simulink model "FinalSolution"  (R2025b)
settings: Solver=VariableStepAuto  StartTime=0.0  StopTime=0.8  FixedStep=SPWM_Ts  RelTol=1e-3
model workspace (MAT data in the model file):
  AC_LoadResistance = 9.23760430703
  AD_TimeConstant = 0.00025
  AD_a = [1 -0.881765205117]
  AD_b = [2.95586987209 -2.95586987209]
  CL_AAComp = 1.00249999972
  CL_Kaw = 20
  CL_Ki = 1.6
  CL_Kp = 0.005
  CL_N = 200
  CL_Ts = 0.0001
  CL_Vref = 32
  CL_faa = 1000
  CL_fp = 50
  CL_mff = 0.94
  CL_mmax = 1
  CommonModeBias = 0.15
  CommonModeKp = 0.02
  CommonModeShift = 1
  ControlStartTime = 0.06
  DampingCapuF = 4.7
  DampingResistance = 30
  DeadtimeComp = 0.08
  DeadtimeCurrentBand = 0.2
  DutyFeedforward = 0
  DutyMax = 0.75
  FilterDCR = 0.3
  KiCurrentLoop = 5
  KiVoltageLoop = 5
  KpCurrentLoop = 0.08
  KpVoltageLoop = 0.2
  LoadConnectTime = 0.18
  MainFilterCapuF = 4.7
  PR_Gain = 1.25
  PR_a10 = [1 -1.99838562653 0.999372033695]
  PR_a11 = [1 -1.99817857535 0.999372066214]
  PR_a13 = [1 -1.99770539603 0.999372140529]
  PR_a16 = [1 -1.99684804391 0.99937227518]
  PR_a17 = [1 -1.99652293757 0.99937232624]
  PR_a19 = [1 -1.9958137982 0.999372437614]
  PR_a2 = [1 -1.99933241937 0.999371884997]
  PR_a4 = [1 -1.99921404574 0.999371903588]
  PR_a5 = [1 -1.99912527012 0.99937191753]
  PR_a7 = [1 -1.9988885544 0.999371954708]
  PR_a8 = [1 -1.99874062131 0.999371977941]
  PR_b10 = [0.236875635534 -0.472442728614 0.23556709308]
  PR_b11 = [0.215389811794 -0.429471148895 0.214081337101]
  PR_b13 = [0.182331988259 -0.363355656682 0.181023668423]
  PR_b16 = [0.148235597863 -0.295163156474 0.146927558611]
  PR_b17 = [0.139542977111 -0.277778021366 0.138235044255]
  PR_b19 = [0.124900915012 -0.248494129248 0.123593214235]
  PR_b2 = [0.425928775502 -0.847596177142 0.42166740164]
  PR_b4 = [0.279572378961 -0.55553023994 0.275957860979]
  PR_b5 = [0.246657018631 -0.490084248228 0.243427229597]
  PR_b7 = [0.202908225742 -0.403457656245 0.200549430503]
  PR_b8 = [0.186290317354 -0.370698545076 0.184408227722]
  PrechargeBypassTime = 0.16
  PrechargeResistance = 47
  RegenerativeMode = 1
  ReturnCurrent = 1.5
  ReturnRampTime = 0.08
  ReturnTs = 1e-05
  SPWM_Ndead = 10
  SPWM_Tdead = 2e-06
  SPWM_Ts = 2e-07
  SPWM_Vgate = 10
  SPWM_f1 = 50
  SPWM_fs = 20000
  SPWM_m = 0.8
  VoltageRampRate = 100
  op_snapshot1 : opcond.OperatingPoint (value not decoded)
  testadd = 0
undefined symbols (not defined in the file): DiscIntNeverNeededParam, dspblkCoreblockFVToolHelper, gcbh
libraries: ee_lib x37, nesl_utility x31, fl_lib x30
(part 2 of 3)

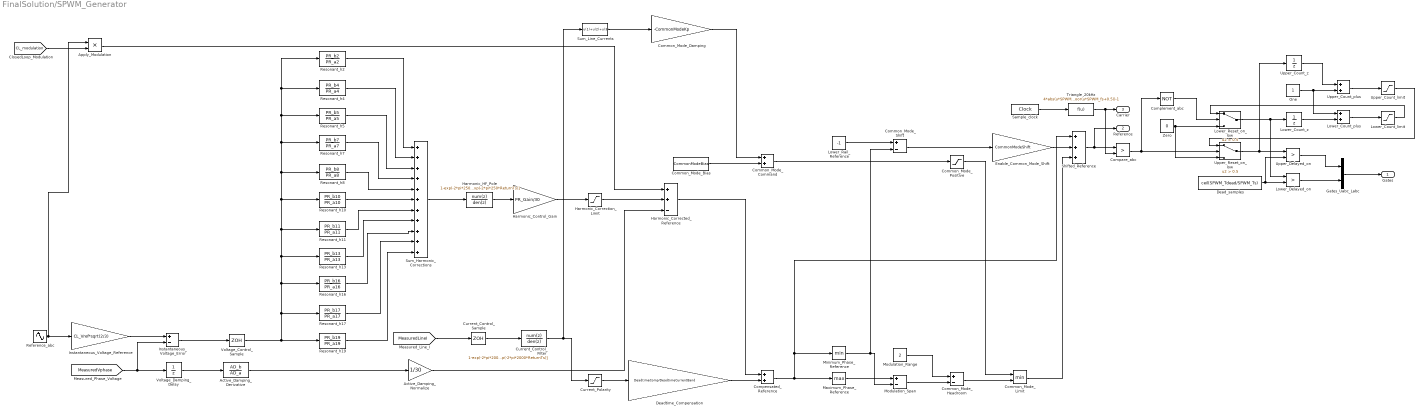
== system FinalSolution/SPWM_Generator ==
  Active_Damping_Derivative : DiscreteTransferFcn  Numerator=AD_b  Denominator=AD_a  SampleTime=ReturnTs
  Active_Damping_Normalize : Gain  Gain=1/30
  Apply_Modulation : Product
  Common_Mode_Bias : Constant  Value=CommonModeBias
  Common_Mode_Command : Sum
  Common_Mode_Damping : Gain  Gain=-CommonModeKp
  Common_Mode_Headroom : Sum  Inputs=+-
  Common_Mode_Limit : MinMax  Inputs=2
  Common_Mode_Positive : Saturate  UpperLimit=2  LowerLimit=0
  Common_Mode_Shift : Sum  Inputs=+-
  Compare_abc : RelationalOperator  Operator=>  OutDataTypeStr=boolean  RndMeth=Simplest  InputSameDT=off
  Compensated_Reference : Sum
  Complement_abc : Logic  Operator=NOT  Inputs=1  IconShape=distinctive  AllPortsSameDT=off  OutDataTypeStr=boolean
  Current_Control_Filter : DiscreteTransferFcn  Numerator=1-exp(-2*pi*2000*ReturnTs)  Denominator=[1 -exp(-2*pi*2000*ReturnTs)]  SampleTime=ReturnTs
  Current_Control_Sample : ZeroOrderHold  SampleTime=ReturnTs
  Current_Polarity : Saturate  UpperLimit=DeadtimeCurrentBand  LowerLimit=-DeadtimeCurrentBand
  Dead_samples : Constant  Value=ceil(SPWM_Tdead/SPWM_Ts)
  Deadtime_Compensation : Gain  Gain=DeadtimeComp/DeadtimeCurrentBand
  Enable_Common_Mode_Shift : Gain  Gain=CommonModeShift
  Gates_Uabc_Labc : Mux  Inputs=2
  Harmonic_Control_Gain : Gain  Gain=PR_Gain/30
  Harmonic_Corrected_Reference : Sum  Inputs=++-
  Harmonic_Correction_Limit : Saturate  UpperLimit=0.15  LowerLimit=-0.15
  Harmonic_HF_Pole : DiscreteTransferFcn  Numerator=1-exp(-2*pi*250*ReturnTs)  Denominator=[1 -exp(-2*pi*250*ReturnTs)]  SampleTime=ReturnTs
  Instantaneous_Voltage_Error : Sum  Inputs=+-
  Instantaneous_Voltage_Reference : Gain  Gain=CL_Vref*sqrt(2/3)
  Lower_Count_limit : Saturate  UpperLimit=ceil(SPWM_Tdead/SPWM_Ts)+1  LowerLimit=0
  Lower_Count_plus : Sum
  Lower_Count_z : UnitDelay  InitialCondition=[0 0 0]  SampleTime=SPWM_Ts  HasFrameUpgradeWarning=on
  Lower_Delayed_on : RelationalOperator  Operator=>  OutDataTypeStr=boolean  RndMeth=Simplest  InputSameDT=off
  Lower_Rail_Reference : Constant  Value=-1
  Lower_Reset_on_low : Switch  Criteria=u2 > Threshold  Threshold=0.5  SaturateOnIntegerOverflow=off  InputSameDT=off
  Maximum_Phase_Reference : MinMax  Function=max
  Minimum_Phase_Reference : MinMax
  Modulation_Range : Constant  Value=2
  Modulation_Span : Sum  Inputs=+-
  One : Constant
  Reference_abc : Sin  Frequency=2*pi*SPWM_f1  Phase=[0 -2*pi/3 2*pi/3]  SampleTime=SPWM_Ts
  Resonant_h10 : DiscreteTransferFcn  Numerator=PR_b10  Denominator=PR_a10  SampleTime=ReturnTs
  Resonant_h11 : DiscreteTransferFcn  Numerator=PR_b11  Denominator=PR_a11  SampleTime=ReturnTs
  Resonant_h13 : DiscreteTransferFcn  Numerator=PR_b13  Denominator=PR_a13  SampleTime=ReturnTs
  Resonant_h16 : DiscreteTransferFcn  Numerator=PR_b16  Denominator=PR_a16  SampleTime=ReturnTs
  Resonant_h17 : DiscreteTransferFcn  Numerator=PR_b17  Denominator=PR_a17  SampleTime=ReturnTs
  Resonant_h19 : DiscreteTransferFcn  Numerator=PR_b19  Denominator=PR_a19  SampleTime=ReturnTs
  Resonant_h2 : DiscreteTransferFcn  Numerator=PR_b2  Denominator=PR_a2  SampleTime=ReturnTs
  Resonant_h4 : DiscreteTransferFcn  Numerator=PR_b4  Denominator=PR_a4  SampleTime=ReturnTs
  Resonant_h5 : DiscreteTransferFcn  Numerator=PR_b5  Denominator=PR_a5  SampleTime=ReturnTs
  Resonant_h7 : DiscreteTransferFcn  Numerator=PR_b7  Denominator=PR_a7  SampleTime=ReturnTs
  Resonant_h8 : DiscreteTransferFcn  Numerator=PR_b8  Denominator=PR_a8  SampleTime=ReturnTs
  Sample_clock : DigitalClock  SampleTime=SPWM_Ts
  Shifted_Reference : Sum  Inputs=+++
  Sum_Harmonic_Corrections : Sum  Inputs=+++++++++++
  Sum_Line_Currents : Fcn  Expr=u(1)+u(2)+u(3)
  Triangle_20kHz : Fcn  Expr=4*abs(u*SPWM_fs-floor(u*SPWM_fs+0.5))-1
  Upper_Count_limit : Saturate  UpperLimit=ceil(SPWM_Tdead/SPWM_Ts)+1  LowerLimit=0
  Upper_Count_plus : Sum
  Upper_Count_z : UnitDelay  InitialCondition=[0 0 0]  SampleTime=SPWM_Ts  HasFrameUpgradeWarning=on
  Upper_Delayed_on : RelationalOperator  Operator=>  OutDataTypeStr=boolean  RndMeth=Simplest  InputSameDT=off
  Upper_Reset_on_low : Switch  Criteria=u2 > Threshold  Threshold=0.5  SaturateOnIntegerOverflow=off  InputSameDT=off
  Voltage_Control_Sample : ZeroOrderHold  SampleTime=ReturnTs
  Voltage_Damping_Delay : UnitDelay  SampleTime=ReturnTs  HasFrameUpgradeWarning=on
  Zero : Constant  Value=0
  Gates : Outport
  Reference : Outport  Port=2
  Carrier : Outport  Port=3
  wires:
  Current_Control_Filter/1 -> Current_Polarity/1, Sum_Line_Currents/1
  Apply_Modulation/1 -> Harmonic_Corrected_Reference/1
  Complement_abc/1 -> Lower_Reset_on_low/2
  [CL_modulation] -> Apply_Modulation/2
  Upper_Count_limit/1 -> Upper_Reset_on_low/1
  Current_Control_Sample/1 -> Current_Control_Filter/1
  Reference_abc/1 -> Apply_Modulation/1, Instantaneous_Voltage_Reference/1
  Zero/1 -> Upper_Reset_on_low/3, Lower_Reset_on_low/3
  Resonant_h10/1 -> Sum_Harmonic_Corrections/6
  Instantaneous_Voltage_Reference/1 -> Instantaneous_Voltage_Error/1
  [MeasuredVphase] -> Voltage_Damping_Delay/1, Instantaneous_Voltage_Error/2
  Instantaneous_Voltage_Error/1 -> Voltage_Control_Sample/1
  Voltage_Control_Sample/1 -> Resonant_h4/1, Resonant_h2/1, Resonant_h5/1, Resonant_h7/1, Resonant_h8/1, Resonant_h10/1, Resonant_h11/1, Resonant_h13/1, Resonant_h16/1, Resonant_h17/1, Resonant_h19/1
  Voltage_Damping_Delay/1 -> Active_Damping_Derivative/1
  Active_Damping_Derivative/1 -> Active_Damping_Normalize/1
  [MeasuredLineI] -> Current_Control_Sample/1
  Resonant_h2/1 -> Sum_Harmonic_Corrections/1
  Harmonic_Corrected_Reference/1 -> Compensated_Reference/1
  Sample_clock/1 -> Triangle_20kHz/1
  Resonant_h4/1 -> Sum_Harmonic_Corrections/2
  Upper_Count_plus/1 -> Upper_Count_limit/1
  Lower_Reset_on_low/1 -> Lower_Count_z/1, Lower_Delayed_on/1
  Resonant_h5/1 -> Sum_Harmonic_Corrections/3
  Gates_Uabc_Labc/1 -> Gates/1
  Resonant_h7/1 -> Sum_Harmonic_Corrections/4
  Resonant_h17/1 -> Sum_Harmonic_Corrections/10
  Resonant_h8/1 -> Sum_Harmonic_Corrections/5
  Resonant_h11/1 -> Sum_Harmonic_Corrections/7
  Resonant_h13/1 -> Sum_Harmonic_Corrections/8
  Lower_Count_plus/1 -> Lower_Count_limit/1
  Compare_abc/1 -> Upper_Reset_on_low/2, Complement_abc/1
  Resonant_h16/1 -> Sum_Harmonic_Corrections/9
  Lower_Rail_Reference/1 -> Common_Mode_Shift/1
  Harmonic_HF_Pole/1 -> Harmonic_Control_Gain/1
  Resonant_h19/1 -> Sum_Harmonic_Corrections/11
  Sum_Harmonic_Corrections/1 -> Harmonic_HF_Pole/1
  Enable_Common_Mode_Shift/1 -> Shifted_Reference/2
  Common_Mode_Positive/1 -> Common_Mode_Limit/1
  Active_Damping_Normalize/1 -> Harmonic_Corrected_Reference/3
  Harmonic_Control_Gain/1 -> Harmonic_Correction_Limit/1
  Sum_Line_Currents/1 -> Common_Mode_Damping/1
  Harmonic_Correction_Limit/1 -> Harmonic_Corrected_Reference/2
  Upper_Reset_on_low/1 -> Upper_Count_z/1, Upper_Delayed_on/1
  Current_Polarity/1 -> Deadtime_Compensation/1
  Dead_samples/1 -> Upper_Delayed_on/2, Lower_Delayed_on/2
  Common_Mode_Damping/1 -> Common_Mode_Command/1
  Common_Mode_Bias/1 -> Common_Mode_Command/2
  Deadtime_Compensation/1 -> Compensated_Reference/2
  Common_Mode_Command/1 -> Common_Mode_Positive/1
  Compensated_Reference/1 -> Shifted_Reference/1, Minimum_Phase_Reference/1, Maximum_Phase_Reference/1
  Minimum_Phase_Reference/1 -> Common_Mode_Shift/2, Modulation_Span/2
  Maximum_Phase_Reference/1 -> Modulation_Span/1
  Common_Mode_Headroom/1 -> Common_Mode_Limit/2
  Common_Mode_Shift/1 -> Enable_Common_Mode_Shift/1
  Common_Mode_Limit/1 -> Shifted_Reference/3
  Modulation_Range/1 -> Common_Mode_Headroom/1
  Modulation_Span/1 -> Common_Mode_Headroom/2
  Triangle_20kHz/1 -> Compare_abc/2, Carrier/1
  Shifted_Reference/1 -> Compare_abc/1, Reference/1
  Lower_Delayed_on/1 -> Gates_Uabc_Labc/2
  Upper_Count_z/1 -> Upper_Count_plus/1
  One/1 -> Upper_Count_plus/2, Lower_Count_plus/1
  Lower_Count_z/1 -> Lower_Count_plus/2
  Upper_Delayed_on/1 -> Gates_Uabc_Labc/1
  Lower_Count_limit/1 -> Lower_Reset_on_low/1

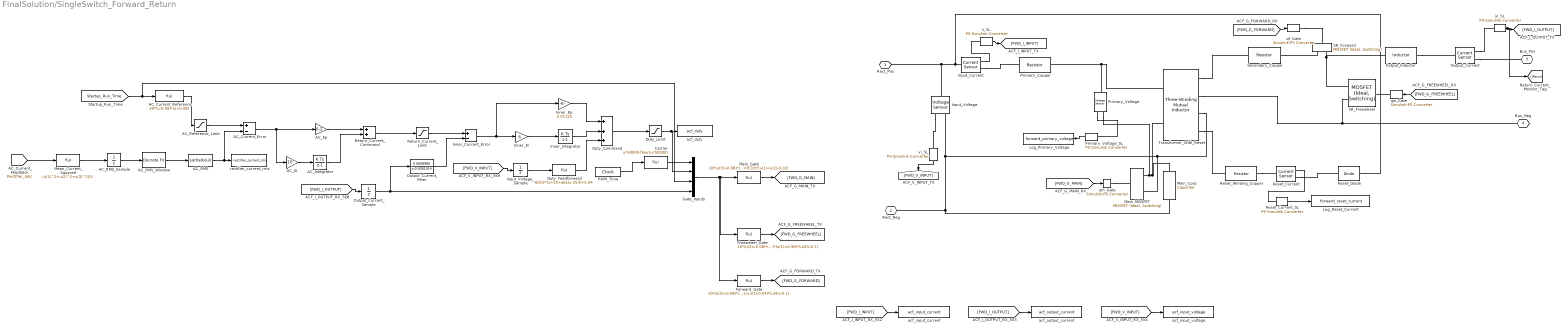
== system FinalSolution/SingleSwitch_Forward_Return ==
  AC_Current_Error : Sum  Inputs=+-
  AC_Current_Reference : Fcn  Expr=20*(u-0.08)*(u>0.08)
  AC_Integrator : DiscreteIntegrator  SampleTime=1e-4  LimitOutput=on  UpperSaturationLimit=2  LowerSaturationLimit=0  ICPrevOutput=DiscIntNeverNeededParam  ICPrevScaledInput=DiscIntNeverNeededParam
  AC_Ki : Gain  Gain=10
  AC_Kp : Gain  Gain=0.2
  AC_RMS : Fcn  Expr=sqrt(abs(u))
  AC_RMS_Sample : UnitDelay  SampleTime=1e-5  HasFrameUpgradeWarning=on
  AC_RMS_Window : DiscreteFir  Coefficients=ones(1,2000)/2000  SampleTime=1e-5
  AC_Reference_Limit : Saturate  UpperLimit=2  LowerLimit=0
  Carrier : Fcn  Expr=u*50000-floor(u*50000)
  Duty_Command : Sum  Inputs=+++
  Duty_Feedforward : Fcn  Expr=60/(2*(u+25+abs(u-25)))+0.04
  Duty_Limit : Saturate  UpperLimit=0.45  LowerLimit=0.02
  Forward_Gate : Fcn  Expr=10*(u(3)>0.08)*(u(1)>0.04)*(u(1)<u(2)-0.04)*(u(4)>0.1)
  Freewheel_Gate : Fcn  Expr=10*(u(3)>0.08)*(u(1)>u(2)+0.04)*(u(1)<0.96)*(u(4)>0.1)
  Gate_Inputs : Mux
  Inner_Current_Error : Sum  Inputs=+-
  Inner_Integrator : DiscreteIntegrator  SampleTime=1e-5  LimitOutput=on  UpperSaturationLimit=0.3  LowerSaturationLimit=-0.3  ICPrevOutput=DiscIntNeverNeededParam  ICPrevScaledInput=DiscIntNeverNeededParam
  Inner_Ki : Gain  Gain=6
  Inner_Kp : Gain  Gain=0.01125
  Input_Current : fl_lib/Electrical/Electrical Sensors/Current Sensor
  Input_Voltage : fl_lib/Electrical/Electrical Sensors/Voltage Sensor
  Input_Voltage_Sample : UnitDelay  SampleTime=1e-5  HasFrameUpgradeWarning=on
  Log_Primary_Voltage : ToWorkspace  VariableName=forward_primary_voltage  SaveFormat=Timeseries  SampleTime=2e-7
  Log_Reset_Current : ToWorkspace  VariableName=forward_reset_current  SaveFormat=Timeseries  SampleTime=2e-7
  Main_Coss : ee_lib/Passive/Capacitor  cap_option=ee.enum.passive.capacitor.capOption.const  c=0.002 uF  Cvec=[1e-05, 1e-06] F  Vvec=[0, 10] V  CV_table_symmetry=ee.enum.passive.capacitor.tableSymmetry.yes  f_vec=[1, 10] kHz  DFext_vec=[.8, 1.2]  enable_C_tol=ee.enum.toleranceApplication.none  averaging_period=0 s  C_tol=5  tol_distribution=ee.enum.toleranceDistribution.uniform  nSigma=4  r=0.1 Ohm  g=0 1/Ohm  enable_operating_limits=ee.enum.enable.no  operating_limit_action=ee.enum.passive.reportOpLim.warn  max_working_voltage_range=[-25, 25] V  power_rating=1 W  maxTemperature=85 degC  thermalEnable=false  thermalMass=1 J/K  i_specify=off  i_priority=None  i=0 A  i_nominal_specify=off  i_nominal_value=1  i_nominal_unit=A  v_specify=off  v_priority=None  v=0 V  v_nominal_specify=off  v_nominal_value=1  v_nominal_unit=V  vc_specify=off  vc_priority=High  vc=0 V  vc_nominal_specify=off  vc_nominal_value=1  vc_nominal_unit=V  T_specify=off  T_priority=None  T=298.15 K  T_nominal_specify=off  T_nominal_value=1  T_nominal_unit=K
  Main_Gate : Fcn  Expr=10*(u(3)>0.08)*(u(1)>=0.02)*(u(1)<u(2)-0.02)
  Main_MOSFET : ee_lib/Semiconductors & Converters/MOSFET (Ideal, Switching)  port_option=ee.enum.controlport.ps  Rds=0.015 Ohm  Goff=1e-6 1/Ohm  Vth=2 V  diode_param=ee.enum.semiconductors.protectionDiode.nodynamics  diode_Vf=0.8 V  diode_Ron=0.001 Ohm  diode_Goff=1e-5 1/Ohm  diode_C=50e-9 F  diode_iRM=-235 A  diode_iF=300 A  diode_idot=-50 A/us  diode_trr_param=ee.enum.converters.diodeReverseParam.trr_factor  diode_trr_factor=3  diode_trr=15 us  diode_Qrr=1500 s*uA  ids_specify=off  ids_priority=None  ids=0 A  ids_nominal_specify=off  ids_nominal_value=1  ids_nominal_unit=A  vds_specify=off  vds_priority=None  vds=0 V  vds_nominal_specify=off  vds_nominal_value=1  vds_nominal_unit=V  vgs_specify=off  vgs_priority=None  vgs=0 V  vgs_nominal_specify=off  vgs_nominal_value=1  vgs_nominal_unit=V  thermal_loss_option=ee.enum.converters.thermalLossOption.constantvalues  Von_data=[0, 1.8, 3.2, 6, 10, 16; 0, 2, 5.5, 9.5, 15, 25] V  Tj=[298.15, 448.15] K  Iout_data=[0, 20, 40, 60, 80, 100] A  Eon_data=[0, 55.04, 124.57, 235.53, 362.12; 0, 71.25, 161.25, 304.88, 468.75] * 1e-6 J  Eoff_data=[0, 18, 30, 56.1, 76.5; 0, 22.5, 37.5, 70.13, 95.63] * 1e-6 J  Eon_data_3D=[zeros(2, 5, 3)] J  Eoff_data_3D=[zeros(2, 5, 3)] J  Tj_loss=[298.15, 448.15] K  Iout_data_loss=[0, 10, 20, 30, 40] A  tabulateWithVds=false  Vds_loss=[0, 150, 300] V  Eon_scalar=22.86e-3 J  Eoff_scalar=17.14e-3 J  Voff=300 V  Iout_scalar=600 A  useCurrentFromPreviousCycle=false  useVoltageFromPreviousCycle=false  diodeModelType=ee.enum.converters.diodeModelType.pwl  diodeTableType=ee.enum.diode.tableType.IfMat  diode_ReverseIVType=ee.enum.diode.diodeReverseIV.constant  diode_IfMat=[.07, .12, .19, 1.75, 4.24, 7.32, 11.2; .16, .3, .72, 2.14, 4.02, 6.35, 9.12] A  diode_VfMat=[.9, 1.15, 1.25, 1.5, 1.75, 2.17, 2.6, 2.85; .58, .68, .75, 1.1, 1.38, 1.77, 2.27, 2.7] V  diode_TjVec=[25, 125] degC  diode_VfVec=[.5, .7, .9, 1.3, 1.7, 2.1, 2.5] V  diode_IfVec=[.1, .2, .5, 1, 2, 4, 7, 10] A  diode_IrMat=[1e-06, 2e-06, 5e-06, 1e-05, 2.5e-05, 5e-05, .0001; 2e-06, 5e-06, 1e-05, 4e-05, 8e-05, .0002, .0005] A  diode_VrMat=[10, 100, 200, 250, 300, 325, 350; 10, 70, 160, 220, 270, 300, 320] V  diode_VrVec=[10, 20, 40, 50, 70, 80, 100] V  diode_IrVec=[1e-06, 2e-06, 5e-06, 1e-05, 2e-05, 5e-05, .0001] A  diode_Vr=-600 V  diode_Ls=150 nH  diode_Erec=0.03 J  diode_rec_loss_model=ee.enum.diode.reverseRecoveryModel.fixed  diode_ErecVal=0 J  diode_scaleWithIandV=true  diode_ErecMat=zeros(2, 3) J  diode_TjrecVec=[298.15, 398.15] K  diode_IfrecVec=[.1, 1, 10] A  diode_IrecVal=10 A  diode_VrecVal=10 V  diode_tFilter=1 / 1000 / 100 s  separateThermalPortForDiode=false  thermal_network_parameterization=ee.enum.thermalNetworkTopology.external  Rth=[.03, .2] K/W  Rth_Cauer=[.03, .1, .2] K/W  Rth_Foster=[.08, .14, .22, .16] K/W  thermal_mass_parameterization=ee.enum.thermalNetwork.timeconstant  thermal_mass=[3, 25] J/K  thermal_mass_Cauer=[3, 10, 25] J/K  thermal_mass_Foster=[.001, .005, .05, .5] J/K  thermal_time_constant=[.1, 5] s  thermal_time_constant_Cauer=[.1, 1, 5] s  thermal_time_constant_Foster=[7e-05, .0007, .01, .08] s  thermal_mass_initial_temperatures=[25, 25] degC  thermal_mass_initial_temperatures_Cauer=[25, 25, 25] degC  junction_thermal_mass=0.1 J/K  Tvec_initial_Foster=[25, 25, 25, 25] degC  RthDiode=[.03, .2] K/W  RthCauerDiode=[.03, .1, .2] K/W  RthFosterDiode=[.03, .2] K/W  thermalMassDiode=[3, 25] J/K  thermalMassCauerDiode=[3, 10, 25] J/K  thermalMassFosterDiode=[33, 50] J/K  thermalTauDiode=[.1, 5] s  thermalTauCauerDiode=[.1, 1, 5] s  thermalTauFosterDiode=[1, 10] s  thermalMassInitTempDiode=[25, 25] degC  thermalMassInitTempCauerDiode=[25, 25, 25] degC  junctionthermalMassDiode=0.1 J/K  TVecInitialFosterDiode=[25, 25, 25, 25] degC  no_thermal_network=0  mosfet_junction_temperature_specify=off  mosfet_junction_temperature_priority=None  mosfet_junction_temperature=25 degC  mosfet_junction_temperature_nominal_specify=off  mosfet_junction_temperature_nominal_value=1  mosfet_junction_temperature_nominal_unit=degC  diode_junction_temperature_specify=off  diode_junction_temperature_priority=None  diode_junction_temperature=25 degC  diode_junction_temperature_nominal_specify=off  diode_junction_temperature_nominal_value=1  diode_junction_temperature_nominal_unit=degC  Qj_specify=off  Qj_priority=None  Qj=0 W  Qj_nominal_specify=off  Qj_nominal_value=1  Qj_nominal_unit=W  accumulatedSwitchingLosses_specify=off  accumulatedSwitchingLosses_priority=None  accumulatedSwitchingLosses=0 J
  Mean_Current_Squared : Fcn  Expr=(u(1)^2+u(2)^2+u(3)^2)/3
  Output_Current : fl_lib/Electrical/Electrical Sensors/Current Sensor
  Output_Current_Filter : DiscreteTransferFcn  Numerator=[0.0608986]  Denominator=[1 -0.9391014]  SampleTime=1e-5
  Output_Current_Sample : UnitDelay  SampleTime=1e-5  HasFrameUpgradeWarning=on
  Output_Inductor : ee_lib/Passive/Inductor  l=2 mH  enable_L_tol=ee.enum.toleranceApplication.none  L_tol=20  tol_distribution=ee.enum.toleranceDistribution.uniform  nSigma=4  r=0.05 Ohm  g=1e-9 1/Ohm  enable_operating_limits=ee.enum.enable.no  operating_limit_action=ee.enum.passive.reportOpLim.warn  max_working_current=1 A  power_rating=1 W  i_L_specify=on  i_L_priority=High  i_L=0 A  i_L_nominal_specify=off  i_L_nominal_value=1  i_L_nominal_unit=A
  PWM_Time : DigitalClock  SampleTime=2e-7
  Primary_Copper : ee_lib/Passive/Resistor  R=0.04 Ohm  enable_R_tol=ee.enum.toleranceApplication.none  R_tol=5  tol_distribution=ee.enum.toleranceDistribution.uniform  nSigma=4  enable_operating_limits=ee.enum.enable.no  operating_limit_action=ee.enum.passive.reportOpLim.warn  power_rating=1 W  max_working_voltage=100 V  noise_mode=ee.enum.sources.noise.Disabled  Tdevice=25 degC  sample_time=1e-3 s  repeatability=ee.enum.ic.repeatability.notRepeatable  user_seed=0  auto_seed=2016017452  power_derating_T1=70 degC  power_derating_T2=155 degC  operating_temperature_range_vec=[-50, 150] degC  alpha=3.93e-3 1/K  Tmeas=25 degC  thermal_mass=100 J/K  temperature_specify=off  temperature_priority=High  temperature=298.15 K  temperature_nominal_specify=off  temperature_nominal_value=1  temperature_nominal_unit=K
  Primary_Voltage : fl_lib/Electrical/Electrical Sensors/Voltage Sensor
  Primary_Voltage_SL : nesl_utility/PS-Simulink Converter  PhysicalDomain=network_engine_domain  SubClassName=ps_output  LeftPortType=input  RightPortType=output  PseudoPeriodic=off  Frequencies=[]  VectorFormat=inherit  Unit=inherit  AffineConversion=off
  Reset_Current : fl_lib/Electrical/Electrical Sensors/Current Sensor
  Reset_Current_SL : nesl_utility/PS-Simulink Converter  PhysicalDomain=network_engine_domain  SubClassName=ps_output  LeftPortType=input  RightPortType=output  PseudoPeriodic=off  Frequencies=[]  VectorFormat=inherit  Unit=inherit  AffineConversion=off
  Reset_Diode : ee_lib/Semiconductors & Converters/Diode  ModelType=ee.enum.diode.modelType.pwl  TableType=ee.enum.diode.tableType.IfMat  IfMat=[.07, .12, .19, 1.75, 4.24, 7.32, 11.2; .16, .3, .72, 2.14, 5.02, 8.35, 13.12] A  VfMat=[.9, 1.15, 1.25, 1.5, 1.75, 2.17, 2.6, 2.85; .58, .68, .75, 1.1, 1.38, 1.77, 2.27, 2.7] V  TjVec=[25, 125] degC  VfVec=[.5, .7, .9, 1.3, 1.7, 2.1, 2.5] V  IfVec=[.1, .2, .5, 1, 2, 4, 7, 10] A  IrMat=[1e-06, 2e-06, 5e-06, 1e-05, 2.5e-05, 5e-05, .0001; 2e-06, 5e-06, 1e-05, 4e-05, 8e-05, .0002, .0005] A  VrMat=[10, 100, 200, 250, 300, 325, 350; 10, 70, 160, 220, 270, 300, 320] V  VrVec=[10, 20, 40, 50, 70, 80, 100] V  IrVec=[1e-06, 2e-06, 5e-06, 1e-05, 2e-05, 5e-05, .0001] A  Vf=0.6 V  Ron=0.3 Ohm  Goff=1e-8 S  prmExp=ee.enum.diode.expParam.useTwo  I12=[.0137, .545] A  V12=[.6, .7] V  RS=0 Ohm  Tmeas=298.15 K  IS=1e-12 A  ec=1  I1=0.0137 A  V1=0.6 V  N_series=1  N_parallel=1  ZenerEnable=false  Rz=0.3 Ohm  BV=inf V  C_param=ee.enum.diode.capParam.fixed  CJ=0 pF  CJ0=5 pF  Vvec=[.1, 10, 100] V  Cvec=[3.5, 1, .4] pF  VJ=1 V  Mgrad=0.5  FC=0.5  Q_param=ee.enum.diode.recoveryParam.off  iRM=-7.15 A  iF=4 A  didt=-750 A/us  trr_factor=3  trr=115 ns  Qrr=150 nA*s  Vr=-600 V  Ls=150 nH  Erec=0.03 J  TT=50 ns  tau=100 ns  T_param=ee.enum.diode.temperatureParam.off  Tdevice=298.15 K  I1_T2=0.245 A  V1_T2=0.5 V  IS_T2=1.25e-7 A  Tmeas2=125 degC  XTI_param=ee.enum.diode.xtiParam.pn  XTI=3  EG_param=ee.enum.diode.egapParam.material_si  EG=1.11 eV  dBVdT=0 V/K  enable_fault_input=simscape.enum.onoff.off  i_specify=off  i_priority=None  i=0 A  i_nominal_specify=off  i_nominal_value=1  i_nominal_unit=A  v_specify=off  v_priority=None  v=0 V  v_nominal_specify=off  v_nominal_value=1  v_nominal_unit=V  v_capacitor_specify=off  v_capacitor_priority=None  v_capacitor=0 V  v_capacitor_nominal_specify=off  v_capacitor_nominal_value=1  v_capacitor_nominal_unit=V  Qj_specify=off  Qj_priority=High  Qj=0 C  Qj_nominal_specify=off  Qj_nominal_value=1  Qj_nominal_unit=C  i_diode_specify=off  i_diode_priority=None  i_diode=0 A  i_diode_nominal_specify=off  i_diode_nominal_value=1  i_diode_nominal_unit=A  v_diode_specify=off  v_diode_priority=None  v_diode=0 V  v_diode_nominal_specify=off  v_diode_nominal_value=1  v_diode_nominal_unit=V  i_capacitor_specify=off  i_capacitor_priority=None  i_capacitor=0 A  i_capacitor_nominal_specify=off  i_capacitor_nominal_value=1  i_capacitor_nominal_unit=A  power_dissipated_specify=off  power_dissipated_priority=None  power_dissipated=0 W  power_dissipated_nominal_specify=off  power_dissipated_nominal_value=1  power_dissipated_nominal_unit=W  fidelity_level=ee.enum.diode.fidelity.includeChargeDyn  rec_loss_model=ee.enum.diode.reverseRecoveryModel.fixed  ErecVal=0 J  scaleWithIandV=true  ErecMat=zeros(2, 3) J  TjrecVec=[298.15, 398.15] K  IfrecVec=[.1, 1, 10] A  IrecVal=10 A  VrecVal=10 V  tFilter=1 / 1000 / 100 s  thermal_network_parameterization=ee.enum.thermalNetworkTopology.junctionCase  Rth=[0, 10] K/W  Rth_Cauer=[1, 3, 10] K/W  Rth_Foster=[.08, .14, .22, .16] K/W  thermal_mass_parameterization=ee.enum.thermalNetwork.timeconstant  thermal_mass=[0, 1] J/K  thermal_mass_Cauer=[.1, .3, 1] J/K  thermal_mass_Foster=[.001, .005, .05, .5] J/K  thermal_time_constant=[0, 10] s  thermal_time_constant_Cauer=[1, 3, 10] s  thermal_time_constant_Foster=[7e-05, .0007, .01, .08] s  thermal_mass_initial_temperatures=[25, 25] degC  thermal_mass_initial_temperatures_Cauer=[25, 25, 25] degC  junction_thermal_mass=0.01 J/K  Tvec_initial_Foster=[25, 25, 25, 25] degC  no_thermal_network=0  junction_temperature_specify=off  junction_temperature_priority=None  junction_temperature=25 degC  junction_temperature_nominal_specify=off  junction_temperature_nominal_value=1  junction_temperature_nominal_unit=degC
  Reset_Winding_Copper : ee_lib/Passive/Resistor  R=0.04 Ohm  enable_R_tol=ee.enum.toleranceApplication.none  R_tol=5  tol_distribution=ee.enum.toleranceDistribution.uniform  nSigma=4  enable_operating_limits=ee.enum.enable.no  operating_limit_action=ee.enum.passive.reportOpLim.warn  power_rating=1 W  max_working_voltage=100 V  noise_mode=ee.enum.sources.noise.Disabled  Tdevice=25 degC  sample_time=1e-3 s  repeatability=ee.enum.ic.repeatability.notRepeatable  user_seed=0  auto_seed=1978802833  power_derating_T1=70 degC  power_derating_T2=155 degC  operating_temperature_range_vec=[-50, 150] degC  alpha=3.93e-3 1/K  Tmeas=25 degC  thermal_mass=100 J/K  temperature_specify=off  temperature_priority=High  temperature=298.15 K  temperature_nominal_specify=off  temperature_nominal_value=1  temperature_nominal_unit=K
  Return_Current_Command : Sum
  Return_Current_Limit : Saturate  UpperLimit=2.2  LowerLimit=0
  SR_Forward : ee_lib/Semiconductors & Converters/MOSFET (Ideal, Switching)  port_option=ee.enum.controlport.ps  Rds=0.015 Ohm  Goff=1e-6 1/Ohm  Vth=2 V  diode_param=ee.enum.semiconductors.protectionDiode.nodynamics  diode_Vf=0.8 V  diode_Ron=0.001 Ohm  diode_Goff=1e-5 1/Ohm  diode_C=50e-9 F  diode_iRM=-235 A  diode_iF=300 A  diode_idot=-50 A/us  diode_trr_param=ee.enum.converters.diodeReverseParam.trr_factor  diode_trr_factor=3  diode_trr=15 us  diode_Qrr=1500 s*uA  ids_specify=off  ids_priority=None  ids=0 A  ids_nominal_specify=off  ids_nominal_value=1  ids_nominal_unit=A  vds_specify=off  vds_priority=None  vds=0 V  vds_nominal_specify=off  vds_nominal_value=1  vds_nominal_unit=V  vgs_specify=off  vgs_priority=None  vgs=0 V  vgs_nominal_specify=off  vgs_nominal_value=1  vgs_nominal_unit=V  thermal_loss_option=ee.enum.converters.thermalLossOption.constantvalues  Von_data=[0, 1.8, 3.2, 6, 10, 16; 0, 2, 5.5, 9.5, 15, 25] V  Tj=[298.15, 448.15] K  Iout_data=[0, 20, 40, 60, 80, 100] A  Eon_data=[0, 55.04, 124.57, 235.53, 362.12; 0, 71.25, 161.25, 304.88, 468.75] * 1e-6 J  Eoff_data=[0, 18, 30, 56.1, 76.5; 0, 22.5, 37.5, 70.13, 95.63] * 1e-6 J  Eon_data_3D=[zeros(2, 5, 3)] J  Eoff_data_3D=[zeros(2, 5, 3)] J  Tj_loss=[298.15, 448.15] K  Iout_data_loss=[0, 10, 20, 30, 40] A  tabulateWithVds=false  Vds_loss=[0, 150, 300] V  Eon_scalar=22.86e-3 J  Eoff_scalar=17.14e-3 J  Voff=300 V  Iout_scalar=600 A  useCurrentFromPreviousCycle=false  useVoltageFromPreviousCycle=false  diodeModelType=ee.enum.converters.diodeModelType.pwl  diodeTableType=ee.enum.diode.tableType.IfMat  diode_ReverseIVType=ee.enum.diode.diodeReverseIV.constant  diode_IfMat=[.07, .12, .19, 1.75, 4.24, 7.32, 11.2; .16, .3, .72, 2.14, 4.02, 6.35, 9.12] A  diode_VfMat=[.9, 1.15, 1.25, 1.5, 1.75, 2.17, 2.6, 2.85; .58, .68, .75, 1.1, 1.38, 1.77, 2.27, 2.7] V  diode_TjVec=[25, 125] degC  diode_VfVec=[.5, .7, .9, 1.3, 1.7, 2.1, 2.5] V  diode_IfVec=[.1, .2, .5, 1, 2, 4, 7, 10] A  diode_IrMat=[1e-06, 2e-06, 5e-06, 1e-05, 2.5e-05, 5e-05, .0001; 2e-06, 5e-06, 1e-05, 4e-05, 8e-05, .0002, .0005] A  diode_VrMat=[10, 100, 200, 250, 300, 325, 350; 10, 70, 160, 220, 270, 300, 320] V  diode_VrVec=[10, 20, 40, 50, 70, 80, 100] V  diode_IrVec=[1e-06, 2e-06, 5e-06, 1e-05, 2e-05, 5e-05, .0001] A  diode_Vr=-600 V  diode_Ls=150 nH  diode_Erec=0.03 J  diode_rec_loss_model=ee.enum.diode.reverseRecoveryModel.fixed  diode_ErecVal=0 J  diode_scaleWithIandV=true  diode_ErecMat=zeros(2, 3) J  diode_TjrecVec=[298.15, 398.15] K  diode_IfrecVec=[.1, 1, 10] A  diode_IrecVal=10 A  diode_VrecVal=10 V  diode_tFilter=1 / 1000 / 100 s  separateThermalPortForDiode=false  thermal_network_parameterization=ee.enum.thermalNetworkTopology.external  Rth=[.03, .2] K/W  Rth_Cauer=[.03, .1, .2] K/W  Rth_Foster=[.08, .14, .22, .16] K/W  thermal_mass_parameterization=ee.enum.thermalNetwork.timeconstant  thermal_mass=[3, 25] J/K  thermal_mass_Cauer=[3, 10, 25] J/K  thermal_mass_Foster=[.001, .005, .05, .5] J/K  thermal_time_constant=[.1, 5] s  thermal_time_constant_Cauer=[.1, 1, 5] s  thermal_time_constant_Foster=[7e-05, .0007, .01, .08] s  thermal_mass_initial_temperatures=[25, 25] degC  thermal_mass_initial_temperatures_Cauer=[25, 25, 25] degC  junction_thermal_mass=0.1 J/K  Tvec_initial_Foster=[25, 25, 25, 25] degC  RthDiode=[.03, .2] K/W  RthCauerDiode=[.03, .1, .2] K/W  RthFosterDiode=[.03, .2] K/W  thermalMassDiode=[3, 25] J/K  thermalMassCauerDiode=[3, 10, 25] J/K  thermalMassFosterDiode=[33, 50] J/K  thermalTauDiode=[.1, 5] s  thermalTauCauerDiode=[.1, 1, 5] s  thermalTauFosterDiode=[1, 10] s  thermalMassInitTempDiode=[25, 25] degC  thermalMassInitTempCauerDiode=[25, 25, 25] degC  junctionthermalMassDiode=0.1 J/K  TVecInitialFosterDiode=[25, 25, 25, 25] degC  no_thermal_network=0  mosfet_junction_temperature_specify=off  mosfet_junction_temperature_priority=None  mosfet_junction_temperature=25 degC  mosfet_junction_temperature_nominal_specify=off  mosfet_junction_temperature_nominal_value=1  mosfet_junction_temperature_nominal_unit=degC  diode_junction_temperature_specify=off  diode_junction_temperature_priority=None  diode_junction_temperature=25 degC  diode_junction_temperature_nominal_specify=off  diode_junction_temperature_nominal_value=1  diode_junction_temperature_nominal_unit=degC  Qj_specify=off  Qj_priority=None  Qj=0 W  Qj_nominal_specify=off  Qj_nominal_value=1  Qj_nominal_unit=W  accumulatedSwitchingLosses_specify=off  accumulatedSwitchingLosses_priority=None  accumulatedSwitchingLosses=0 J
  SR_Freewheel : ee_lib/Semiconductors & Converters/MOSFET (Ideal, Switching)  port_option=ee.enum.controlport.ps  Rds=0.015 Ohm  Goff=1e-6 1/Ohm  Vth=2 V  diode_param=ee.enum.semiconductors.protectionDiode.nodynamics  diode_Vf=0.8 V  diode_Ron=0.001 Ohm  diode_Goff=1e-5 1/Ohm  diode_C=50e-9 F  diode_iRM=-235 A  diode_iF=300 A  diode_idot=-50 A/us  diode_trr_param=ee.enum.converters.diodeReverseParam.trr_factor  diode_trr_factor=3  diode_trr=15 us  diode_Qrr=1500 s*uA  ids_specify=off  ids_priority=None  ids=0 A  ids_nominal_specify=off  ids_nominal_value=1  ids_nominal_unit=A  vds_specify=off  vds_priority=None  vds=0 V  vds_nominal_specify=off  vds_nominal_value=1  vds_nominal_unit=V  vgs_specify=off  vgs_priority=None  vgs=0 V  vgs_nominal_specify=off  vgs_nominal_value=1  vgs_nominal_unit=V  thermal_loss_option=ee.enum.converters.thermalLossOption.constantvalues  Von_data=[0, 1.8, 3.2, 6, 10, 16; 0, 2, 5.5, 9.5, 15, 25] V  Tj=[298.15, 448.15] K  Iout_data=[0, 20, 40, 60, 80, 100] A  Eon_data=[0, 55.04, 124.57, 235.53, 362.12; 0, 71.25, 161.25, 304.88, 468.75] * 1e-6 J  Eoff_data=[0, 18, 30, 56.1, 76.5; 0, 22.5, 37.5, 70.13, 95.63] * 1e-6 J  Eon_data_3D=[zeros(2, 5, 3)] J  Eoff_data_3D=[zeros(2, 5, 3)] J  Tj_loss=[298.15, 448.15] K  Iout_data_loss=[0, 10, 20, 30, 40] A  tabulateWithVds=false  Vds_loss=[0, 150, 300] V  Eon_scalar=22.86e-3 J  Eoff_scalar=17.14e-3 J  Voff=300 V  Iout_scalar=600 A  useCurrentFromPreviousCycle=false  useVoltageFromPreviousCycle=false  diodeModelType=ee.enum.converters.diodeModelType.pwl  diodeTableType=ee.enum.diode.tableType.IfMat  diode_ReverseIVType=ee.enum.diode.diodeReverseIV.constant  diode_IfMat=[.07, .12, .19, 1.75, 4.24, 7.32, 11.2; .16, .3, .72, 2.14, 4.02, 6.35, 9.12] A  diode_VfMat=[.9, 1.15, 1.25, 1.5, 1.75, 2.17, 2.6, 2.85; .58, .68, .75, 1.1, 1.38, 1.77, 2.27, 2.7] V  diode_TjVec=[25, 125] degC  diode_VfVec=[.5, .7, .9, 1.3, 1.7, 2.1, 2.5] V  diode_IfVec=[.1, .2, .5, 1, 2, 4, 7, 10] A  diode_IrMat=[1e-06, 2e-06, 5e-06, 1e-05, 2.5e-05, 5e-05, .0001; 2e-06, 5e-06, 1e-05, 4e-05, 8e-05, .0002, .0005] A  diode_VrMat=[10, 100, 200, 250, 300, 325, 350; 10, 70, 160, 220, 270, 300, 320] V  diode_VrVec=[10, 20, 40, 50, 70, 80, 100] V  diode_IrVec=[1e-06, 2e-06, 5e-06, 1e-05, 2e-05, 5e-05, .0001] A  diode_Vr=-600 V  diode_Ls=150 nH  diode_Erec=0.03 J  diode_rec_loss_model=ee.enum.diode.reverseRecoveryModel.fixed  diode_ErecVal=0 J  diode_scaleWithIandV=true  diode_ErecMat=zeros(2, 3) J  diode_TjrecVec=[298.15, 398.15] K  diode_IfrecVec=[.1, 1, 10] A  diode_IrecVal=10 A  diode_VrecVal=10 V  diode_tFilter=1 / 1000 / 100 s  separateThermalPortForDiode=false  thermal_network_parameterization=ee.enum.thermalNetworkTopology.external  Rth=[.03, .2] K/W  Rth_Cauer=[.03, .1, .2] K/W  Rth_Foster=[.08, .14, .22, .16] K/W  thermal_mass_parameterization=ee.enum.thermalNetwork.timeconstant  thermal_mass=[3, 25] J/K  thermal_mass_Cauer=[3, 10, 25] J/K  thermal_mass_Foster=[.001, .005, .05, .5] J/K  thermal_time_constant=[.1, 5] s  thermal_time_constant_Cauer=[.1, 1, 5] s  thermal_time_constant_Foster=[7e-05, .0007, .01, .08] s  thermal_mass_initial_temperatures=[25, 25] degC  thermal_mass_initial_temperatures_Cauer=[25, 25, 25] degC  junction_thermal_mass=0.1 J/K  Tvec_initial_Foster=[25, 25, 25, 25] degC  RthDiode=[.03, .2] K/W  RthCauerDiode=[.03, .1, .2] K/W  RthFosterDiode=[.03, .2] K/W  thermalMassDiode=[3, 25] J/K  thermalMassCauerDiode=[3, 10, 25] J/K  thermalMassFosterDiode=[33, 50] J/K  thermalTauDiode=[.1, 5] s  thermalTauCauerDiode=[.1, 1, 5] s  thermalTauFosterDiode=[1, 10] s  thermalMassInitTempDiode=[25, 25] degC  thermalMassInitTempCauerDiode=[25, 25, 25] degC  junctionthermalMassDiode=0.1 J/K  TVecInitialFosterDiode=[25, 25, 25, 25] degC  no_thermal_network=0  mosfet_junction_temperature_specify=off  mosfet_junction_temperature_priority=None  mosfet_junction_temperature=25 degC  mosfet_junction_temperature_nominal_specify=off  mosfet_junction_temperature_nominal_value=1  mosfet_junction_temperature_nominal_unit=degC  diode_junction_temperature_specify=off  diode_junction_temperature_priority=None  diode_junction_temperature=25 degC  diode_junction_temperature_nominal_specify=off  diode_junction_temperature_nominal_value=1  diode_junction_temperature_nominal_unit=degC  Qj_specify=off  Qj_priority=None  Qj=0 W  Qj_nominal_specify=off  Qj_nominal_value=1  Qj_nominal_unit=W  accumulatedSwitchingLosses_specify=off  accumulatedSwitchingLosses_priority=None  accumulatedSwitchingLosses=0 J
  Secondary_Copper : ee_lib/Passive/Resistor  R=0.06 Ohm  enable_R_tol=ee.enum.toleranceApplication.none  R_tol=5  tol_distribution=ee.enum.toleranceDistribution.uniform  nSigma=4  enable_operating_limits=ee.enum.enable.no  operating_limit_action=ee.enum.passive.reportOpLim.warn  power_rating=1 W  max_working_voltage=100 V  noise_mode=ee.enum.sources.noise.Disabled  Tdevice=25 degC  sample_time=1e-3 s  repeatability=ee.enum.ic.repeatability.notRepeatable  user_seed=0  auto_seed=51119000  power_derating_T1=70 degC  power_derating_T2=155 degC  operating_temperature_range_vec=[-50, 150] degC  alpha=3.93e-3 1/K  Tmeas=25 degC  thermal_mass=100 J/K  temperature_specify=off  temperature_priority=High  temperature=298.15 K  temperature_nominal_specify=off  temperature_nominal_value=1  temperature_nominal_unit=K
  Transformer_With_Reset : ee_lib/Passive/Transformers/Three-Winding Mutual Inductor  L1=0.002 H  L2=0.032 H  L3=0.002 H  perfectCoupling=false  K12=0.9998  K13=0.9998  K23=0.9998  i1_specify=on  i1_priority=High  i1=0 A  i1_nominal_specify=off  i1_nominal_value=1  i1_nominal_unit=A  i2_specify=on  i2_priority=High  i2=0 A  i2_nominal_specify=off  i2_nominal_value=1  i2_nominal_unit=A  i3_specify=on  i3_priority=High  i3=0 A  i3_nominal_specify=off  i3_nominal_value=1  i3_nominal_unit=A
      settings: InternalSimscapePortConfiguration="{\"Bottom\":[],\"Left\":[{\"id\":\"p1\",\"label\":\"1+\",\"type\":\"foundation.electrical.electrical\"},{\"id\":\"n1\",\"label\":\"1-\",\"type\":\"foundation.electrical.electrical\"}],\"Right\":[{\"id\":\"p2\",\"label\":\"2+\",\"type\":\"foundation.electrical.electrical\"},{\"id\":\"n2\",\"label\":\"2-\",\"type\":\"foundation.electrical.electrical\"},{\"id\":\"p3\",\"label\":\"3+\",\"type\":\"foundation.electrical.electrical\"},{\"id\":\"n3\",\"label\":\"3-\",\"type\":\"foundation.electrical.electrical\"}],\"Top\":[]}"
  acf_duty : ToWorkspace  VariableName=acf_duty  SaveFormat=Timeseries  SampleTime=1e-5
  acf_input_current : ToWorkspace  VariableName=acf_input_current  SaveFormat=Timeseries  SampleTime=2e-7
  acf_input_voltage : ToWorkspace  VariableName=acf_input_voltage  SaveFormat=Timeseries  SampleTime=2e-7
  acf_output_current : ToWorkspace  VariableName=acf_output_current  SaveFormat=Timeseries  SampleTime=2e-7
  ii_SL : nesl_utility/PS-Simulink Converter  PhysicalDomain=network_engine_domain  SubClassName=ps_output  LeftPortType=input  RightPortType=output  PseudoPeriodic=off  Frequencies=[]  VectorFormat=inherit  Unit=inherit  AffineConversion=off
  io_SL : nesl_utility/PS-Simulink Converter  PhysicalDomain=network_engine_domain  SubClassName=ps_output  LeftPortType=input  RightPortType=output  PseudoPeriodic=off  Frequencies=[]  VectorFormat=inherit  Unit=inherit  AffineConversion=off
  qf_Gate : nesl_utility/Simulink-PS Converter  PhysicalDomain=network_engine_domain  SubClassName=ps_input  LeftPortType=input  RightPortType=output  PseudoPeriodic=off  Frequencies=[]  NoiseDistribution=none  NoiseParameters=[]  Unit=1  AffineConversion=off  FilteringAndDerivatives=provide  SimscapeFilterOrder=1  InputFilterTimeConstant=0.001  UdotUserProvided=0
  qm_Gate : nesl_utility/Simulink-PS Converter  PhysicalDomain=network_engine_domain  SubClassName=ps_input  LeftPortType=input  RightPortType=output  PseudoPeriodic=off  Frequencies=[]  NoiseDistribution=none  NoiseParameters=[]  Unit=1  AffineConversion=off  FilteringAndDerivatives=provide  SimscapeFilterOrder=1  InputFilterTimeConstant=0.001  UdotUserProvided=0
  qw_Gate : nesl_utility/Simulink-PS Converter  PhysicalDomain=network_engine_domain  SubClassName=ps_input  LeftPortType=input  RightPortType=output  PseudoPeriodic=off  Frequencies=[]  NoiseDistribution=none  NoiseParameters=[]  Unit=1  AffineConversion=off  FilteringAndDerivatives=provide  SimscapeFilterOrder=1  InputFilterTimeConstant=0.001  UdotUserProvided=0
  rectifier_current_rms : ToWorkspace  VariableName=rectifier_current_rms  SaveFormat=Timeseries  SampleTime=1e-5
  vi_SL : nesl_utility/PS-Simulink Converter  PhysicalDomain=network_engine_domain  SubClassName=ps_output  LeftPortType=input  RightPortType=output  PseudoPeriodic=off  Frequencies=[]  VectorFormat=inherit  Unit=inherit  AffineConversion=off
  Rect_Pos : PMIOPort  Side=Left
  Rect_Neg : PMIOPort  Port=2  Side=Left
  Bus_Pos : PMIOPort  Port=3  Side=Right
  Bus_Neg : PMIOPort  Port=4  Side=Right
  tag scope: I_Return=global
  wires:
  Carrier/1 -> Gate_Inputs/1
  Inner_Integrator/1 -> Duty_Command/2
  Output_Current_Filter/1 -> Inner_Current_Error/2
  AC_Integrator/1 -> Return_Current_Command/2
  Duty_Limit/1 -> Gate_Inputs/2, acf_duty/1
  Gate_Inputs/1 -> Freewheel_Gate/1, Main_Gate/1, Forward_Gate/1
  Duty_Command/1 -> Duty_Limit/1
  Inner_Kp/1 -> Duty_Command/1
  Inner_Ki/1 -> Inner_Integrator/1
  Inner_Current_Error/1 -> Inner_Kp/1, Inner_Ki/1
  Return_Current_Limit/1 -> Inner_Current_Error/1
  Return_Current_Command/1 -> Return_Current_Limit/1
  AC_Kp/1 -> Return_Current_Command/1
  AC_Ki/1 -> AC_Integrator/1
  AC_Current_Error/1 -> AC_Kp/1, AC_Ki/1
  AC_Reference_Limit/1 -> AC_Current_Error/1
  PWM_Time/1 -> Carrier/1
  [FWD_V_INPUT] -> acf_input_voltage/1
  [FWD_V_INPUT] -> Input_Voltage_Sample/1
  [FWD_I_OUTPUT] -> acf_output_current/1
  [FWD_I_OUTPUT] -> Output_Current_Sample/1
  [FWD_I_INPUT] -> acf_input_current/1
  [FWD_G_FREEWHEEL] -> qw_Gate/1
  Freewheel_Gate/1 -> [FWD_G_FREEWHEEL]
  [FWD_G_FORWARD] -> qf_Gate/1
  Forward_Gate/1 -> [FWD_G_FORWARD]
  [FWD_G_MAIN] -> qm_Gate/1
  Main_Gate/1 -> [FWD_G_MAIN]
  AC_RMS_Sample/1 -> AC_RMS_Window/1
  Mean_Current_Squared/1 -> AC_RMS_Sample/1
  Input_Voltage_Sample/1 -> Duty_Feedforward/1
  Output_Current_Sample/1 -> Gate_Inputs/4, Output_Current_Filter/1
  [Rectifier_Iabc] -> Mean_Current_Squared/1
  AC_RMS_Window/1 -> AC_RMS/1
  vi_SL/1 -> [FWD_V_INPUT]
  ii_SL/1 -> [FWD_I_INPUT]
  AC_RMS/1 -> AC_Current_Error/2, rectifier_current_rms/1
  Duty_Feedforward/1 -> Duty_Command/3
  Primary_Voltage_SL/1 -> Log_Primary_Voltage/1
  Reset_Current_SL/1 -> Log_Reset_Current/1
  io_SL/1 -> [FWD_I_OUTPUT], [I_Return]
  [Startup_Run_Time] -> AC_Current_Reference/1, Gate_Inputs/3
  AC_Current_Reference/1 -> AC_Reference_Limit/1
  connections:
  SR_Freewheel/RConn1 -- Output_Inductor/LConn1 -- SR_Forward/RConn1
  Output_Inductor/RConn1 -- Output_Current/LConn1
  Output_Current/RConn2 -- Bus_Pos/RConn1
  qw_Gate/RConn1 -- SR_Freewheel/LConn1
  qf_Gate/RConn1 -- SR_Forward/LConn1
  Output_Current/RConn1 -- io_SL/LConn1
  Primary_Voltage/RConn1 -- Primary_Voltage_SL/LConn1
  Reset_Current/RConn1 -- Reset_Current_SL/LConn1
  Reset_Current/RConn2 -- Reset_Diode/LConn1
  Reset_Winding_Copper/RConn1 -- Reset_Current/LConn1
  Transformer_With_Reset/RConn4 -- Reset_Winding_Copper/LConn1
  Transformer_With_Reset/RConn1 -- Secondary_Copper/LConn1
  Primary_Voltage/LConn1 -- Primary_Copper/RConn1 -- Transformer_With_Reset/LConn1
  Transformer_With_Reset/RConn2 -- Bus_Neg/RConn1 -- SR_Freewheel/RConn2
  Transformer_With_Reset/LConn2 -- Main_MOSFET/RConn1 -- Primary_Voltage/RConn2 -- Main_Coss/LConn1
  Input_Current/RConn1 -- ii_SL/LConn1
  Input_Voltage/RConn1 -- vi_SL/LConn1
  qm_Gate/RConn1 -- Main_MOSFET/LConn1
  Secondary_Copper/RConn1 -- SR_Forward/RConn2
  Transformer_With_Reset/RConn3 -- Rect_Neg/RConn1 -- Main_Coss/RConn1 -- Input_Voltage/RConn2 -- Main_MOSFET/RConn2
  Input_Current/RConn2 -- Primary_Copper/LConn1
  Rect_Pos/RConn1 -- Reset_Diode/RConn1 -- Input_Current/LConn1 -- Input_Voltage/LConn1

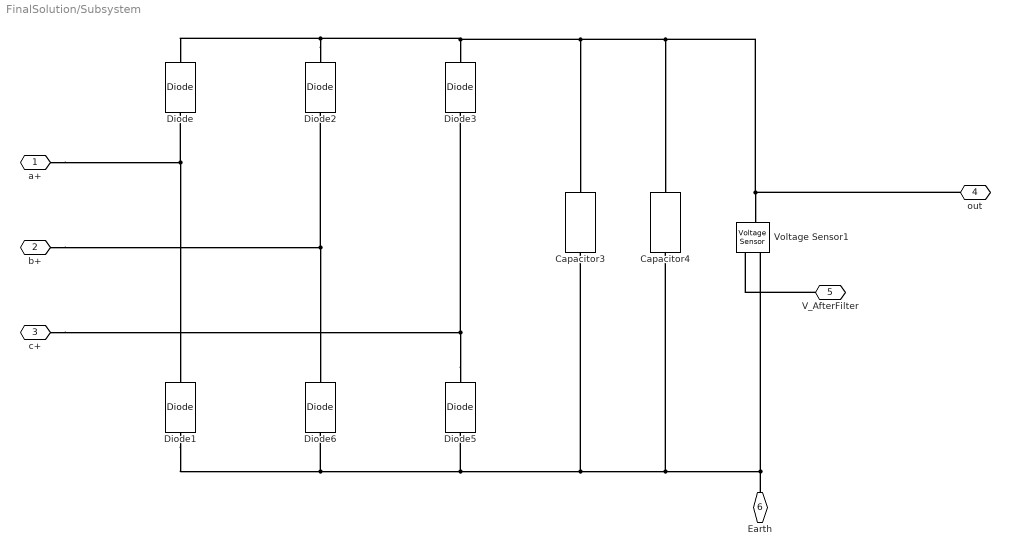
== system FinalSolution/Subsystem ==
  Capacitor3 : ee_lib/Passive/Capacitor  cap_option=ee.enum.passive.capacitor.capOption.const  c=1 uF  Cvec=[1e-05, 1e-06] F  Vvec=[0, 10] V  CV_table_symmetry=ee.enum.passive.capacitor.tableSymmetry.yes  f_vec=[1, 10] kHz  DFext_vec=[.8, 1.2]  enable_C_tol=ee.enum.toleranceApplication.none  averaging_period=0 s  C_tol=5  tol_distribution=ee.enum.toleranceDistribution.uniform  nSigma=4  r=0.1 Ohm  g=0 1/Ohm  enable_operating_limits=ee.enum.enable.no  operating_limit_action=ee.enum.passive.reportOpLim.warn  max_working_voltage_range=[-25, 25] V  power_rating=1 W  maxTemperature=85 degC  thermalEnable=false  thermalMass=1 J/K  i_specify=off  i_priority=None  i=0 A  i_nominal_specify=off  i_nominal_value=1  i_nominal_unit=A  v_specify=off  v_priority=None  v=0 V  v_nominal_specify=off  v_nominal_value=1  v_nominal_unit=V  vc_specify=on  vc_priority=High  vc=0 V  vc_nominal_specify=off  vc_nominal_value=1  vc_nominal_unit=V  T_specify=off  T_priority=None  T=298.15 K  T_nominal_specify=off  T_nominal_value=1  T_nominal_unit=K
  Capacitor4 : ee_lib/Passive/Capacitor  cap_option=ee.enum.passive.capacitor.capOption.const  c=470 uF  Cvec=[1e-05, 1e-06] F  Vvec=[0, 10] V  CV_table_symmetry=ee.enum.passive.capacitor.tableSymmetry.yes  f_vec=[1, 10] kHz  DFext_vec=[.8, 1.2]  enable_C_tol=ee.enum.toleranceApplication.none  averaging_period=0 s  C_tol=5  tol_distribution=ee.enum.toleranceDistribution.uniform  nSigma=4  r=0.1 Ohm  g=0 1/Ohm  enable_operating_limits=ee.enum.enable.no  operating_limit_action=ee.enum.passive.reportOpLim.warn  max_working_voltage_range=[-25, 25] V  power_rating=1 W  maxTemperature=85 degC  thermalEnable=false  thermalMass=1 J/K  i_specify=off  i_priority=None  i=0 A  i_nominal_specify=off  i_nominal_value=1  i_nominal_unit=A  v_specify=off  v_priority=None  v=0 V  v_nominal_specify=off  v_nominal_value=1  v_nominal_unit=V  vc_specify=on  vc_priority=High  vc=0 V  vc_nominal_specify=off  vc_nominal_value=1  vc_nominal_unit=V  T_specify=off  T_priority=None  T=298.15 K  T_nominal_specify=off  T_nominal_value=1  T_nominal_unit=K
  Diode{,1..3,5..6} (6 alike) : ee_lib/Semiconductors & Converters/Diode  ModelType=ee.enum.diode.modelType.pwl  TableType=ee.enum.diode.tableType.IfMat  IfMat=[.07, .12, .19, 1.75, 4.24, 7.32, 11.2; .16, .3, .72, 2.14, 5.02, 8.35, 13.12] A  VfMat=[.9, 1.15, 1.25, 1.5, 1.75, 2.17, 2.6, 2.85; .58, .68, .75, 1.1, 1.38, 1.77, 2.27, 2.7] V  TjVec=[25, 125] degC  VfVec=[.5, .7, .9, 1.3, 1.7, 2.1, 2.5] V  IfVec=[.1, .2, .5, 1, 2, 4, 7, 10] A  IrMat=[1e-06, 2e-06, 5e-06, 1e-05, 2.5e-05, 5e-05, .0001; 2e-06, 5e-06, 1e-05, 4e-05, 8e-05, .0002, .0005] A  VrMat=[10, 100, 200, 250, 300, 325, 350; 10, 70, 160, 220, 270, 300, 320] V  VrVec=[10, 20, 40, 50, 70, 80, 100] V  IrVec=[1e-06, 2e-06, 5e-06, 1e-05, 2e-05, 5e-05, .0001] A  Vf=0.6 V  Ron=0.3 Ohm  Goff=1e-8 S  prmExp=ee.enum.diode.expParam.useTwo  I12=[.0137, .545] A  V12=[.6, .7] V  RS=0 Ohm  Tmeas=298.15 K  IS=1e-12 A  ec=1  I1=0.0137 A  V1=0.6 V  N_series=1  N_parallel=1  ZenerEnable=false  Rz=0.3 Ohm  BV=inf V  C_param=ee.enum.diode.capParam.fixed  CJ=0 pF  CJ0=5 pF  Vvec=[.1, 10, 100] V  Cvec=[3.5, 1, .4] pF  VJ=1 V  Mgrad=0.5  FC=0.5  Q_param=ee.enum.diode.recoveryParam.off  iRM=-7.15 A  iF=4 A  didt=-750 A/us  trr_factor=3  trr=115 ns  Qrr=150 nA*s  Vr=-600 V  Ls=150 nH  Erec=0.03 J  TT=50 ns  tau=100 ns  T_param=ee.enum.diode.temperatureParam.off  Tdevice=298.15 K  I1_T2=0.245 A  V1_T2=0.5 V  IS_T2=1.25e-7 A  Tmeas2=125 degC  XTI_param=ee.enum.diode.xtiParam.pn  XTI=3  EG_param=ee.enum.diode.egapParam.material_si  EG=1.11 eV  dBVdT=0 V/K  enable_fault_input=simscape.enum.onoff.off  i_specify=off  i_priority=None  i=0 A  i_nominal_specify=off  i_nominal_value=1  i_nominal_unit=A  v_specify=off  v_priority=None  v=0 V  v_nominal_specify=off  v_nominal_value=1  v_nominal_unit=V  v_capacitor_specify=off  v_capacitor_priority=None  v_capacitor=0 V  v_capacitor_nominal_specify=off  v_capacitor_nominal_value=1  v_capacitor_nominal_unit=V  Qj_specify=off  Qj_priority=High  Qj=0 C  Qj_nominal_specify=off  Qj_nominal_value=1  Qj_nominal_unit=C  i_diode_specify=off  i_diode_priority=None  i_diode=0 A  i_diode_nominal_specify=off  i_diode_nominal_value=1  i_diode_nominal_unit=A  v_diode_specify=off  v_diode_priority=None  v_diode=0 V  v_diode_nominal_specify=off  v_diode_nominal_value=1  v_diode_nominal_unit=V  i_capacitor_specify=off  i_capacitor_priority=None  i_capacitor=0 A  i_capacitor_nominal_specify=off  i_capacitor_nominal_value=1  i_capacitor_nominal_unit=A  power_dissipated_specify=off  power_dissipated_priority=None  power_dissipated=0 W  power_dissipated_nominal_specify=off  power_dissipated_nominal_value=1  power_dissipated_nominal_unit=W  fidelity_level=ee.enum.diode.fidelity.includeChargeDyn  rec_loss_model=ee.enum.diode.reverseRecoveryModel.fixed  ErecVal=0 J  scaleWithIandV=true  ErecMat=zeros(2, 3) J  TjrecVec=[298.15, 398.15] K  IfrecVec=[.1, 1, 10] A  IrecVal=10 A  VrecVal=10 V  tFilter=1 / 1000 / 100 s  thermal_network_parameterization=ee.enum.thermalNetworkTopology.junctionCase  Rth=[0, 10] K/W  Rth_Cauer=[1, 3, 10] K/W  Rth_Foster=[.08, .14, .22, .16] K/W  thermal_mass_parameterization=ee.enum.thermalNetwork.timeconstant  thermal_mass=[0, 1] J/K  thermal_mass_Cauer=[.1, .3, 1] J/K  thermal_mass_Foster=[.001, .005, .05, .5] J/K  thermal_time_constant=[0, 10] s  thermal_time_constant_Cauer=[1, 3, 10] s  thermal_time_constant_Foster=[7e-05, .0007, .01, .08] s  thermal_mass_initial_temperatures=[25, 25] degC  thermal_mass_initial_temperatures_Cauer=[25, 25, 25] degC  junction_thermal_mass=0.01 J/K  Tvec_initial_Foster=[25, 25, 25, 25] degC  no_thermal_network=0  junction_temperature_specify=off  junction_temperature_priority=None  junction_temperature=25 degC  junction_temperature_nominal_specify=off  junction_temperature_nominal_value=1  junction_temperature_nominal_unit=degC
  Voltage Sensor1 : fl_lib/Electrical/Electrical Sensors/Voltage Sensor
  a+ : PMIOPort  Side=Left
  b+ : PMIOPort  Port=2  Side=Left
  c+ : PMIOPort  Port=3  Side=Left
  out : PMIOPort  Port=4  Side=Right
  V_AfterFilter : PMIOPort  Port=5  Side=Right
  Earth : PMIOPort  Port=6  Side=Right
  connections:
  Diode5/RConn1 -- c+/RConn1 -- Diode3/LConn1
  Diode2/RConn1 -- out/RConn1 -- Voltage Sensor1/LConn1 -- Capacitor4/LConn1 -- Capacitor3/LConn1 -- Diode3/RConn1 -- Diode/RConn1
  Diode2/LConn1 -- b+/RConn1 -- Diode6/RConn1
  Diode/LConn1 -- a+/RConn1 -- Diode1/RConn1
  V_AfterFilter/RConn1 -- Voltage Sensor1/RConn1
  Diode6/LConn1 -- Capacitor3/RConn1 -- Capacitor4/RConn1 -- Voltage Sensor1/RConn2 -- Earth/RConn1 -- Diode5/LConn1 -- Diode1/LConn1
